simulink model "kcat_tv"  (Simulink 5.0)
settings: Solver=ode45  StartTime=0.0  StopTime=100.0  RelTol=1e-3
values from neighbouring files (symbols this model uses):
  H = [1 0]    [constant_velocity.m]    (also in damposc.m; harmosc_ricatti.mat; harmosc_riccati.mat; kf_resistor_demo.m = 1)
  I = [1  0; 0  1]    [harmosc_ricatti.mat]    (also in harmosc_riccati.mat; kalgen.m = eye(n); lec.m = ones(n,1); state9.m = eye(n))
  P0 = [0.01 0; 0 0.01]    [constant_velocity.m]    (also in damposc.m; harmosc_ricatti.mat = [0.95  0; 0  1]; harmosc_riccati.mat = [1  0; 0  1]; kalgen.m = proc_noise * eye(n))
  Q = [0.0001 0; 0 0.000001]    [constant_velocity.m]    (also in damposc.m = [0.00001 0; 0 0.000001]; harmosc_ricatti.mat = [1  0; 0  1]; harmosc_riccati.mat = [1  0; 0  1]; kalgen.m = proc_noise * eye(n))
  R = Re + h    (= 6378441.8)    [Ainit.m]    (also in constant_velocity.m = 1; damposc.m = 0.01; harmosc_ricatti.mat = 2; harmosc_riccati.mat = 3)
undefined symbols (not defined in the file or in its folder): rss_ratio, ud_inv
libraries: simulink x2
settings Model: Creator=mcar  LastModifiedBy=mcarroll  ExtModeAutoUpdateStatusClock=off  LoadExternalInput=on  ExternalInput=[inStruct]  SaveFormat=StructureWithTime  OptimizeBlockIOStorage=off

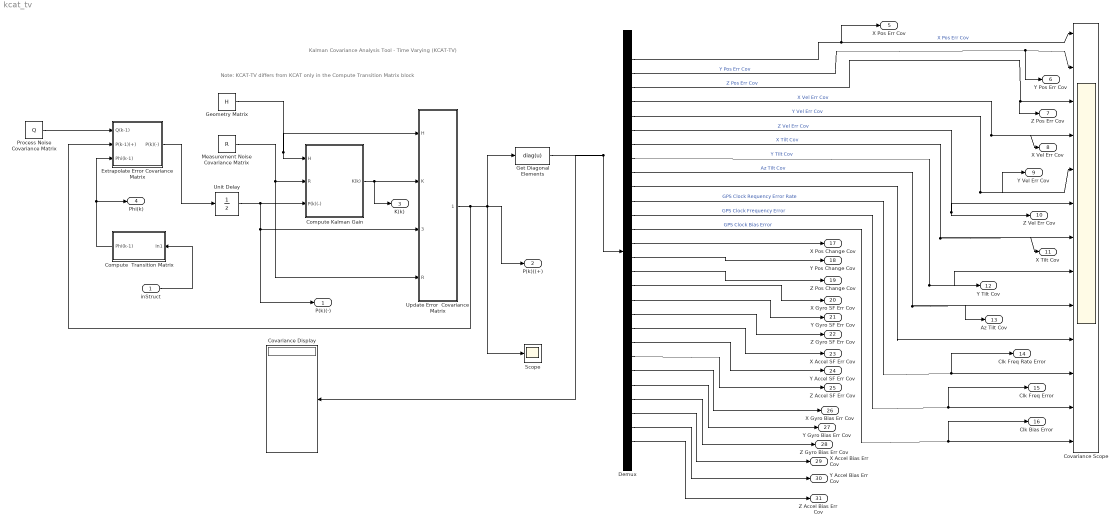
== system kcat_tv ==
  note: Kalman Covariance Analysis Tool - Time Varying
      | (KCAT-TV)
  note: Note:  KCAT-TV differs from KCAT only in the
      | Compute Transition Matrix block
  inStruct : Inport  PortDimensions=[28 28]
  Compute  Transition Matrix : Subsystem  Orientation=left
  Compute Kalman Gain : Subsystem
  Covariance Display : Display
  Covariance Scope : Scope  NumInputPorts=13
      settings: TimeRange=10  YMin=-20~-5~-5~-5~-5~-5~-5~-5~-5~-5~-5~-5~-5  YMax=120~5~5~5~5~5~5~5~5~5~5~5~5  SaveName=ScopeData11
  Demux : Demux  Outputs=28
  Extrapolate Error Covariance Matrix : Subsystem
  Geometry Matrix : Constant  Value=H  VectorParams1D=off
  Get Diagonal Elements : MATLABFcn  MATLABFcn=diag(u)  Output1D=off
  Measurement Noise Covariance Matrix : Constant  Value=R  VectorParams1D=off  ShowAdditionalParam=on
  Process Noise Covariance Matrix : Constant  Value=Q  VectorParams1D=off
  Scope : Scope
      settings: TimeRange=10  YMin=-20  YMax=120  SaveName=ScopeData4
  Unit Delay : UnitDelay  X0=P0
  Update Error  Covariance Matrix : Subsystem
  P(k)(-) : Outport
  P(k)((+) : Outport  Port=2
  K(k) : Outport  Port=3
  Phi(k) : Outport  Port=4
  X Pos Err Cov : Outport  Port=5
  Y Pos Err Cov : Outport  Port=6
  Z Pos Err Cov : Outport  Port=7
  X Vel Err Cov : Outport  Port=8
  Y Vel Err Cov : Outport  Port=9
  Z Vel Err Cov : Outport  Port=10
  X Tilt Cov : Outport  Port=11
  Y Tilt Cov : Outport  Port=12
  Az Tilt Cov : Outport  Port=13
  Clk Freq Rate Error : Outport  Port=14
  Clk Freq Error : Outport  Port=15
  Clk Bias Error : Outport  Port=16
  X Pos Change Cov : Outport  Port=17
  Y Pos Change Cov : Outport  Port=18
  Z Pos Change Cov : Outport  Port=19
  X Gyro SF Err Cov : Outport  Port=20
  Y Gyro SF Err Cov : Outport  Port=21
  Z Gyro SF Err Cov : Outport  Port=22
  X Accel SF Err Cov : Outport  Port=23
  Y Accel SF Err Cov : Outport  Port=24
  Z Accel SF Err Cov : Outport  Port=25
  X Gyro Bias Err Cov : Outport  Port=26
  Y Gyro Bias Err Cov : Outport  Port=27
  Z Gyro Bias Err Cov : Outport  Port=28
  X Accel Bias Err Cov : Outport  Port=29
  Y Accel Bias Err Cov : Outport  Port=30
  Z Accel Bias Err Cov : Outport  Port=31
  wires:
  Update Error  Covariance Matrix/1(P(k)(+)) -> P(k)((+)/1, Scope/1, Get Diagonal Elements/1, Extrapolate Error Covariance Matrix/2(P(k-1)(+))
  Unit Delay/1 -> Compute Kalman Gain/3(P(k)(-)), Update Error  Covariance Matrix/3(P(k)(-)), P(k)(-)/1
  Compute Kalman Gain/1(K(k)) -> Update Error  Covariance Matrix/2(K), K(k)/1
  Process Noise Covariance Matrix/1 -> Extrapolate Error Covariance Matrix/1(Q(k-1))
  Extrapolate Error Covariance Matrix/1(P(k)(-)) -> Unit Delay/1
  Compute  Transition Matrix/1(Phi(k-1)) -> Extrapolate Error Covariance Matrix/3(Phi(k-1)), Phi(k)/1
  Geometry Matrix/1 -> Compute Kalman Gain/1(H), Update Error  Covariance Matrix/1(H)
  Measurement Noise Covariance Matrix/1 -> Compute Kalman Gain/2(R), Update Error  Covariance Matrix/4(R)
  inStruct/1 -> Compute  Transition Matrix/1(In1)
  Get Diagonal Elements/1 -> Covariance Display/1, Demux/1
  Demux/9 -> Covariance Scope/9, Az Tilt Cov/1  "Az Tilt Cov"
  Demux/8 -> Covariance Scope/8, Y Tilt Cov/1  "Y Tilt Cov"
  Demux/7 -> Covariance Scope/7, X Tilt Cov/1  "X Tilt Cov"
  Demux/6 -> Covariance Scope/6, Z Vel Err Cov/1  "Z Vel Err Cov"
  Demux/5 -> Covariance Scope/5, Y Vel Err Cov/1  "Y Vel Err Cov"
  Demux/4 -> Covariance Scope/4, X Vel Err Cov/1  "X Vel Err Cov"
  Demux/3 -> Covariance Scope/3, Z Pos Err Cov/1  "Z Pos Err Cov"
  Demux/1 -> Covariance Scope/1, X Pos Err Cov/1  "X Pos Err Cov"
  Demux/10 -> Covariance Scope/10
  Demux/11 -> Covariance Scope/11, Clk Freq Rate Error/1  "GPS Clock Requency Error Rate"
  Demux/12 -> Covariance Scope/12, Clk Freq Error/1  "GPS Clock Frequency Error"
  Demux/13 -> Covariance Scope/13, Clk Bias Error/1  "GPS Clock Bias Error"
  Demux/2 -> Covariance Scope/2, Y Pos Err Cov/1  "Y Pos Err Cov"
  Demux/14 -> X Pos Change Cov/1
  Demux/15 -> Y Pos Change Cov/1
  Demux/16 -> Z Pos Change Cov/1
  Demux/17 -> X Gyro SF Err Cov/1
  Demux/18 -> Y Gyro SF Err Cov/1
  Demux/19 -> Z Gyro SF Err Cov/1
  Demux/20 -> X Accel SF Err Cov/1
  Demux/21 -> Y Accel SF Err Cov/1
  Demux/22 -> Z Accel SF Err Cov/1
  Demux/23 -> X Gyro Bias Err Cov/1
  Demux/24 -> Y Gyro Bias Err Cov/1
  Demux/25 -> Z Gyro Bias Err Cov/1
  Demux/26 -> X Accel Bias Err Cov/1
  Demux/27 -> Y Accel Bias Err Cov/1
  Demux/28 -> Z Accel Bias Err Cov/1

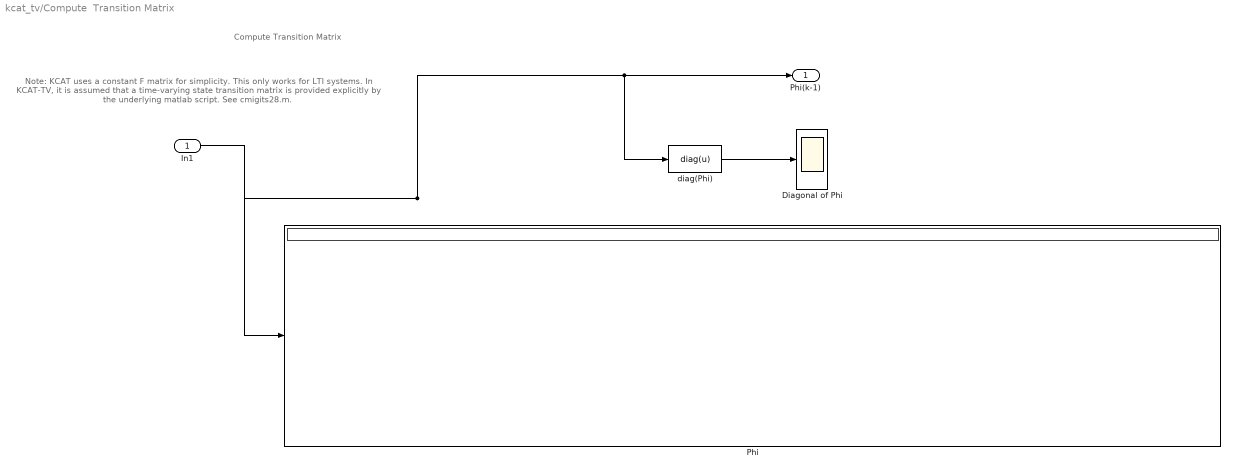
== system kcat_tv/Compute  Transition Matrix ==
  note: Compute Transition Matrix
  note: Note:  KCAT uses a constant F matrix
      | for simplicity.  This only works for LTI
      | systems.  In KCAT-TV, it is assumed that a
      | time-varying state transition matrix is provided
      | explicitly by the underlying matlab script.  See
      | cmigits28.m.
  In1 : Inport
  Diagonal of Phi : Scope
      settings: YMin=0  YMax=2  SaveName=ScopeData3
  Phi : Display
  diag(Phi) : MATLABFcn  MATLABFcn=diag(u)
  Phi(k-1) : Outport
  wires:
  In1/1 -> Phi/1, Phi(k-1)/1, diag(Phi)/1
  diag(Phi)/1 -> Diagonal of Phi/1

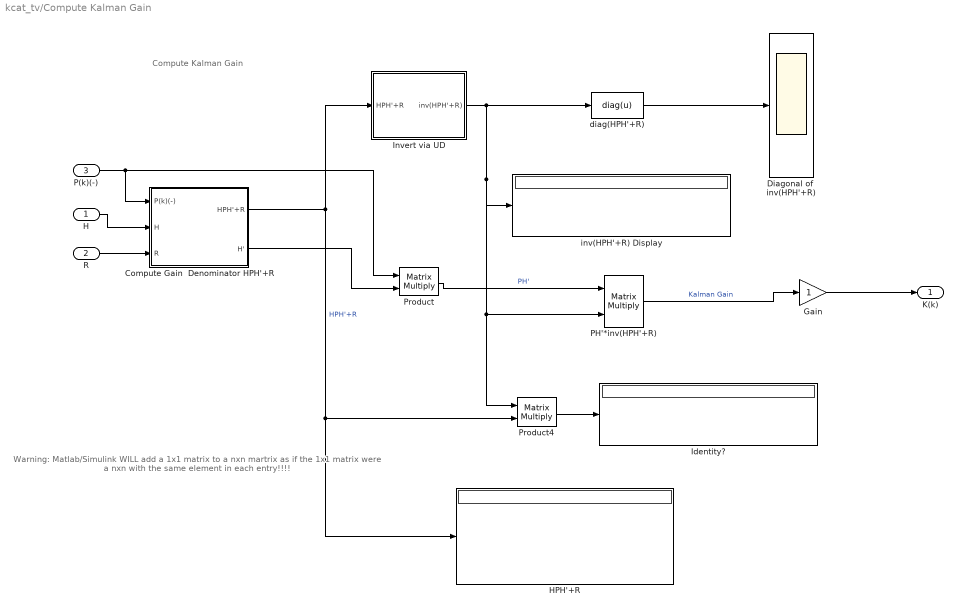
== system kcat_tv/Compute Kalman Gain ==
  note: Compute Kalman Gain
  note: Warning:
      | Matlab/Simulink
      | WILL add a 1x1 matrix to
      | a nxn martrix as if the
      | 1x1 matrix were a
      | nxn with the same element
      | in each entry!!!!
  H : Inport
  R : Inport  Port=2
  P(k)(-) : Inport  Port=3  ShowAdditionalParam=on
  Compute Gain  Denominator HPH'+R : Subsystem
  Diagonal of  inv(HPH'+R) : Scope
      settings: TimeRange=100  YMin=0.0006  YMax=0.002  SaveName=ScopeData2
  Gain : Gain  ShowAdditionalParam=on  SaturateOnIntegerOverflow=on
  HPH'+R : Display
  Identity? : Display
  Invert via UD : Subsystem
  PH'*inv(HPH'+R) : Product  Multiplication=Matrix(*)  ShowAdditionalParam=on
  Product : Product  Multiplication=Matrix(*)  SaturateOnIntegerOverflow=on
  Product4 : Product  Multiplication=Matrix(*)  ShowAdditionalParam=on  SaturateOnIntegerOverflow=on  InputSameDT=on
  diag(HPH'+R) : MATLABFcn  MATLABFcn=diag(u)
  inv(HPH'+R) Display : Display
  K(k) : Outport
  wires:
  Compute Gain  Denominator HPH'+R/1(HPH'+R) -> Invert via UD/1(HPH'+R), HPH'+R/1, Product4/2  "HPH'+R"
  R/1 -> Compute Gain  Denominator HPH'+R/3(R)
  diag(HPH'+R)/1 -> Diagonal of  inv(HPH'+R)/1
  Invert via UD/1(inv(HPH'+R)) -> diag(HPH'+R)/1, inv(HPH'+R) Display/1, PH'*inv(HPH'+R)/2, Product4/1
  Compute Gain  Denominator HPH'+R/2(H') -> Product/2
  Product/1 -> PH'*inv(HPH'+R)/1  "PH'"
  Product4/1 -> Identity?/1
  H/1 -> Compute Gain  Denominator HPH'+R/2(H)
  P(k)(-)/1 -> Compute Gain  Denominator HPH'+R/1(P(k)(-)), Product/1
  PH'*inv(HPH'+R)/1 -> Gain/1  "Kalman Gain"
  Gain/1 -> K(k)/1

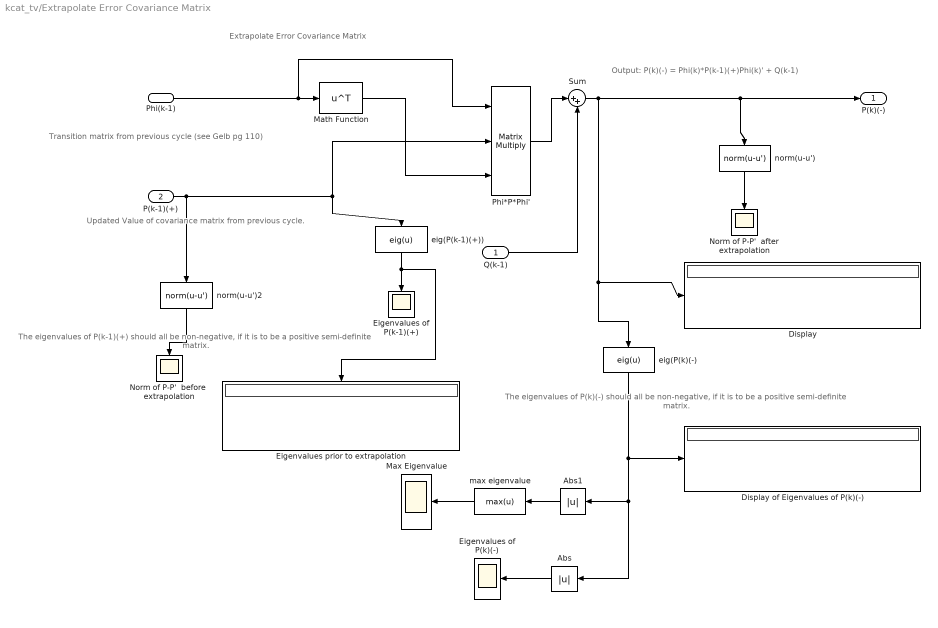
== system kcat_tv/Extrapolate Error Covariance Matrix ==
  note: The eigenvalues of P(k)(-) should all be non-negative,
      | if it is to be a positive semi-definite matrix.
  note: The eigenvalues of P(k-1)(+) should all be
      | non-negative, if it is to be a positive
      | semi-definite matrix.
  note: Transition matrix from
      | previous cycle
      | (see Gelb pg 110)
  note: Output: P(k)(-) = Phi(k)*P(k-1)(+)Phi(k)' + Q(k-1)
  note: Updated Value of
      | covariance matrix  from
      | previous cycle.
  note: Extrapolate Error Covariance Matrix
  Q(k-1) : Inport
  P(k-1)(+) : Inport  Port=2
  Phi(k-1) : Inport  Port=3
  Abs : Abs  Orientation=left  SaturateOnIntegerOverflow=on
  Abs1 : Abs  Orientation=left  SaturateOnIntegerOverflow=on
  Display : Display
  Display of Eigenvalues of P(k)(-) : Display
  Eigenvalues prior to extrapolation : Display
      settings: Orientation=down
  Eigenvalues of P(k)(-) : Scope
      settings: SaveName=ScopeData8
  Eigenvalues of P(k-1)(+) : Scope
      settings: Orientation=down  YMin=1  YMax=8.5  SaveName=ScopeData7
  Math Function : Math  Operator=transpose
  Max Eigenvalue : Scope
      settings: TimeRange=100  YMin=0  YMax=4e+072  SaveName=ScopeData12
  Norm of P-P'  after extrapolation : Scope
      settings: Orientation=down  TimeRange=10  YMin=0  YMax=35  SaveName=ScopeData15
  Norm of P-P'  before  extrapolation : Scope
      settings: Orientation=down  TimeRange=10  YMin=0  YMax=35  SaveName=ScopeData16
  Phi*P*Phi' : Product  Inputs=3  Multiplication=Matrix(*)  SaturateOnIntegerOverflow=on  InputSameDT=on
  Sum : Sum  Inputs=|++  SaturateOnIntegerOverflow=on  InputSameDT=on
  eig(P(k)(-) : MATLABFcn  Orientation=down  MATLABFcn=eig(u)  OutputSignalType=complex
  eig(P(k-1)(+)) : MATLABFcn  Orientation=down  MATLABFcn=eig(u)
  max eigenvalue : MATLABFcn  Orientation=left  MATLABFcn=max(u)  Output1D=off
  norm(u-u') : MATLABFcn  Orientation=down  MATLABFcn=norm(u-u')  Output1D=off
  norm(u-u')2 : MATLABFcn  Orientation=down  MATLABFcn=norm(u-u')  Output1D=off
  P(k)(-) : Outport
  wires:
  Math Function/1 -> Phi*P*Phi'/3
  max eigenvalue/1 -> Max Eigenvalue/1
  Abs1/1 -> max eigenvalue/1
  Abs/1 -> Eigenvalues of P(k)(-)/1
  norm(u-u')2/1 -> Norm of P-P'  before  extrapolation/1
  norm(u-u')/1 -> Norm of P-P'  after extrapolation/1
  eig(P(k)(-)/1 -> Abs1/1, Abs/1, Display of Eigenvalues of P(k)(-)/1
  eig(P(k-1)(+))/1 -> Eigenvalues prior to extrapolation/1, Eigenvalues of P(k-1)(+)/1
  Q(k-1)/1 -> Sum/2
  P(k-1)(+)/1 -> Phi*P*Phi'/2, eig(P(k-1)(+))/1, norm(u-u')2/1
  Phi(k-1)/1 -> Phi*P*Phi'/1, Math Function/1
  Sum/1 -> norm(u-u')/1, P(k)(-)/1, eig(P(k)(-)/1, Display/1
  Phi*P*Phi'/1 -> Sum/1

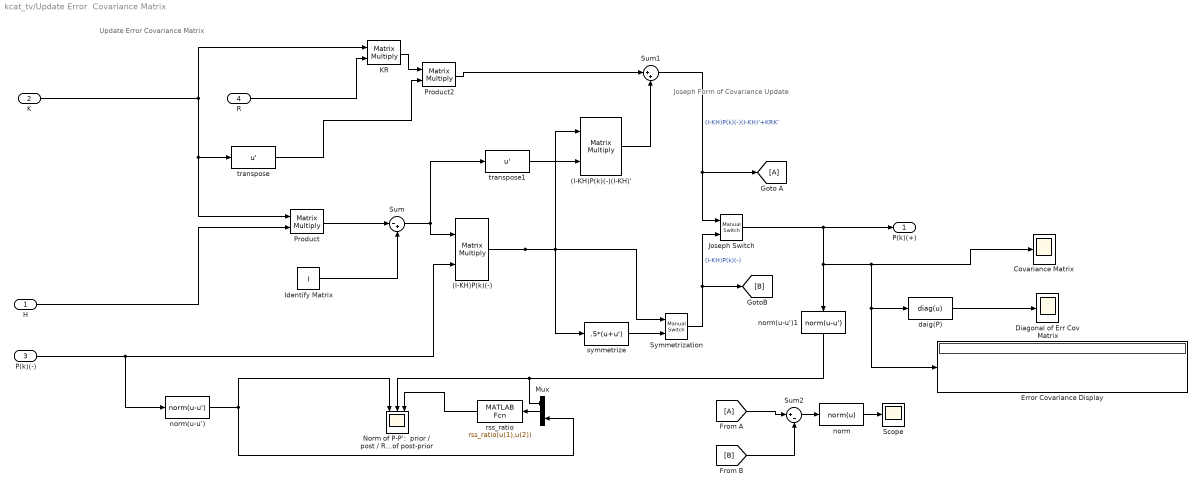
== system kcat_tv/Update Error  Covariance Matrix ==
  note: Update Error Covariance Matrix
  note: Joseph Form
      | of Covariance
      | Update
  H : Inport
  K : Inport  Port=2  ShowAdditionalParam=on
  P(k)(-) : Inport  Port=3
  R : Inport  Port=4
  (I-KH)P(k)(-) : Product  Multiplication=Matrix(*)  SaturateOnIntegerOverflow=on  InputSameDT=on
  (I-KH)P(k)(-)(I-KH)' : Product  Multiplication=Matrix(*)  SaturateOnIntegerOverflow=on  InputSameDT=on
  Covariance Matrix : Scope
      settings: TimeRange=10  YMin=-60  YMax=80
  Diagonal of Err Cov Matrix : Scope
      settings: YMin=0  YMax=5000
  Error Covariance Display : Display
  Identify Matrix : Constant  Value=I  VectorParams1D=off
  Joseph Switch : simulink/Signal Routing/Manual Switch  sw=1  action=0
  KR : Product  Multiplication=Matrix(*)  SaturateOnIntegerOverflow=on
  Mux : Mux  Orientation=left  Inputs=2
  Norm of P-P':  prior / post / RSS ratio of post-prior : Scope  NumInputPorts=3
      settings: Orientation=down  TimeRange=10  YMin=0~0~0  YMax=40~2~0.05  SaveName=ScopeData13
  Product : Product  Multiplication=Matrix(*)  SaturateOnIntegerOverflow=on  InputSameDT=on
  Product2 : Product  Multiplication=Matrix(*)  SaturateOnIntegerOverflow=on
  Scope : Scope
      settings: SaveName=ScopeData14
  Sum : Sum  Inputs=|-+  SaturateOnIntegerOverflow=on  InputSameDT=on
  Sum1 : Sum  Inputs=|++  SaturateOnIntegerOverflow=on  InputSameDT=on
  Sum2 : Sum  Inputs=|+-  SaturateOnIntegerOverflow=on  InputSameDT=on
  Symmetrization : simulink/Signal Routing/Manual Switch  sw=1  action=0
  daig(P) : MATLABFcn  MATLABFcn=diag(u)
  norm : MATLABFcn  MATLABFcn=norm(u)  Output1D=off
  norm(u-u') : MATLABFcn  MATLABFcn=norm(u-u')  Output1D=off
  norm(u-u')1 : MATLABFcn  Orientation=down  MATLABFcn=norm(u-u')  Output1D=off
  rss_ratio : MATLABFcn  Orientation=left  MATLABFcn=rss_ratio(u(1),u(2))  OutputSignalType=real
  symmetrize : MATLABFcn  MATLABFcn=.5*(u+u')  Output1D=off
  transpose : MATLABFcn  MATLABFcn=u'  Output1D=off
  transpose1 : MATLABFcn  MATLABFcn=u'  Output1D=off
  P(k)(+) : Outport
  wires:
  H/1 -> Product/2
  K/1 -> Product/1, transpose/1, KR/1
  P(k)(-)/1 -> (I-KH)P(k)(-)/2, norm(u-u')/1
  Identify Matrix/1 -> Sum/2
  Product/1 -> Sum/1
  Sum/1 -> (I-KH)P(k)(-)/1, transpose1/1
  R/1 -> KR/2
  transpose/1 -> Product2/2
  (I-KH)P(k)(-)/1 -> (I-KH)P(k)(-)(I-KH)'/1, Symmetrization/1, symmetrize/1
  transpose1/1 -> (I-KH)P(k)(-)(I-KH)'/2
  (I-KH)P(k)(-)(I-KH)'/1 -> Sum1/2
  Product2/1 -> Sum1/1
  symmetrize/1 -> Symmetrization/2
  Symmetrization/1 -> Joseph Switch/2, [B]  "(I-KH)P(k)(-)"
  Joseph Switch/1 -> P(k)(+)/1, norm(u-u')1/1, daig(P)/1, Error Covariance Display/1, Covariance Matrix/1
  Sum1/1 -> Joseph Switch/1, [A]  "(I-KH)P(k)(-)(I-KH)'+KRK'"
  norm(u-u')/1 -> Norm of P-P':  prior / post / RSS ratio of post-prior/1, Mux/2
  norm(u-u')1/1 -> Norm of P-P':  prior / post / RSS ratio of post-prior/2, Mux/1
  rss_ratio/1 -> Norm of P-P':  prior / post / RSS ratio of post-prior/3
  Mux/1 -> rss_ratio/1
  [B] -> Sum2/2
  [A] -> Sum2/1
  Sum2/1 -> norm/1
  norm/1 -> Scope/1
  daig(P)/1 -> Diagonal of Err Cov Matrix/1
  KR/1 -> Product2/1

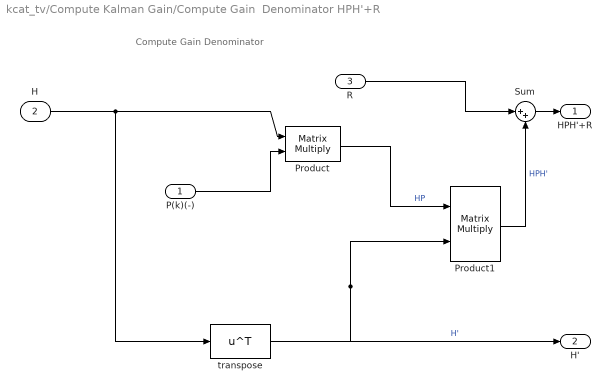
== system kcat_tv/Compute Kalman Gain/Compute Gain  Denominator HPH'+R ==
  note: Compute Gain Denominator
  P(k)(-) : Inport
  H : Inport  Port=2
  R : Inport  Port=3
  Product : Product  Multiplication=Matrix(*)  SaturateOnIntegerOverflow=on  InputSameDT=on
  Product1 : Product  Multiplication=Matrix(*)  ShowAdditionalParam=on  SaturateOnIntegerOverflow=on
  Sum : Sum  Inputs=|++  ShowAdditionalParam=on  SaturateOnIntegerOverflow=on  InputSameDT=on
  transpose : Math  Operator=transpose
  HPH'+R : Outport
  H' : Outport  Port=2
  wires:
  transpose/1 -> H'/1, Product1/2  "H'"
  Product1/1 -> Sum/2  "HPH'"
  Product/1 -> Product1/1  "HP"
  H/1 -> Product/1, transpose/1
  R/1 -> Sum/1
  Sum/1 -> HPH'+R/1
  P(k)(-)/1 -> Product/2

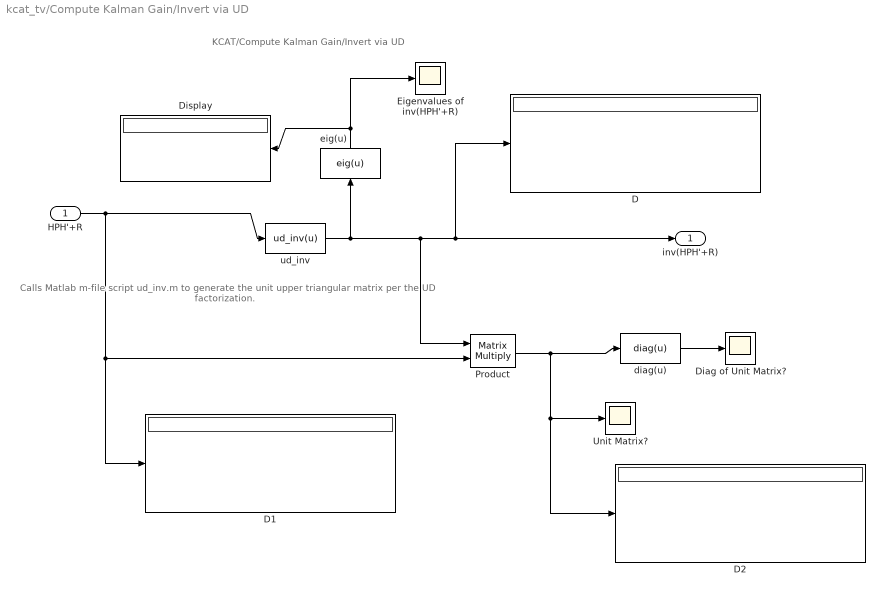
== system kcat_tv/Compute Kalman Gain/Invert via UD ==
  note: Calls Matlab m-file script ud_inv.m
      | to generate the unit upper triangular
      | matrix per the UD factorization.
  note: KCAT/Compute Kalman Gain/Invert via UD
  HPH'+R : Inport
  D : Display
  D1 : Display
  D2 : Display
  Diag of Unit Matrix? : Scope
      settings: YMin=0.99  YMax=1.03  SaveName=ScopeData10
  Display : Display
  Eigenvalues of inv(HPH'+R) : Scope
      settings: SaveName=ScopeData6
  Product : Product  Multiplication=Matrix(*)  SaturateOnIntegerOverflow=on  InputSameDT=on
  Unit Matrix? : Scope
      settings: SaveName=ScopeData9
  diag(u) : MATLABFcn  MATLABFcn=diag(u)  Output1D=off
  eig(u) : MATLABFcn  Orientation=up  MATLABFcn=eig(u)  Output1D=off
  ud_inv : MATLABFcn  MATLABFcn=ud_inv(u)  Output1D=off
  inv(HPH'+R) : Outport
  wires:
  HPH'+R/1 -> ud_inv/1, D1/1, Product/2
  ud_inv/1 -> eig(u)/1, inv(HPH'+R)/1, D/1, Product/1
  eig(u)/1 -> Eigenvalues of inv(HPH'+R)/1, Display/1
  Product/1 -> diag(u)/1, Unit Matrix?/1, D2/1
  diag(u)/1 -> Diag of Unit Matrix?/1
